simulink model "dofstuff"  (R2026b)
settings: Solver=ode4  StopTime=60  FixedStep=0.01
values from neighbouring files (symbols this model uses):
  dragCoeffVec = [CdAx;CdAy;CdAz]    [init_quadrotor.m]
  g = params.g    [QuadrotorEOM.m]    (also in QuadrotorPlant.m; init_quadrotor.m = 9.81)
  Kdtheta = 15.0    (= 15)    [init_quadrotor.m]
  Kdz = 60.0    (= 60)    [init_quadrotor.m]
  Kitheta = 5.0    (= 5)    [init_quadrotor.m]
  Kiz = 0.0    (= 0)    [init_quadrotor.m]
  Kptheta = 20.0    (= 20)    [init_quadrotor.m]
  Kpz = 150.0    (= 150)    [init_quadrotor.m]
  m = 256    [PlotAircraftSim.m]    (also in QuadrotorEOM.m = params.m; QuadrotorPlant.m = params.m; init_quadrotor.m = 5.6)
  rho = 1.225    [init_quadrotor.m]
libraries: aerolibfltsims x2, aerolibanimutils x1
settings Model: SimulationMode=accelerator  Creator=YoYo  LastModifiedBy=YoYo
settings SolverCC: MinimalZcImpactIntegration=on
settings DataIOCC: DSMLogging=off  ReturnWorkspaceOutputs=off  SaveOutput=off  SaveTime=off  SignalLogging=off
settings DebuggingCC: MultiTaskDSMMsg=none  ReadBeforeWriteMsg=DisableAll  WriteAfterReadMsg=DisableAll  WriteAfterWriteMsg=DisableAll
settings SFSimCC: SFSimEcho=off

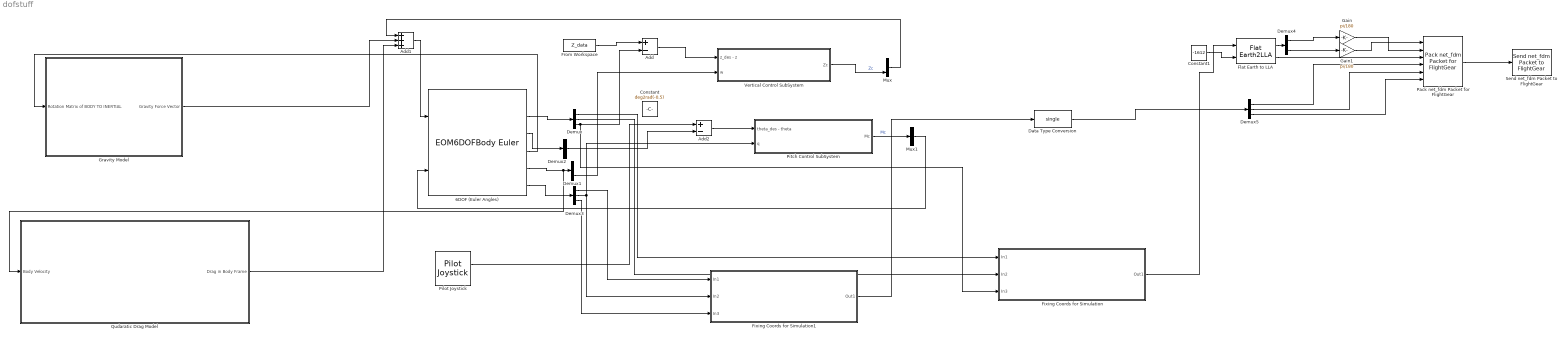
== system dofstuff ==
  6DOF (Euler Angles) : EOM6DOFBodyEuler  mass_0=5.6
  Add : Sum  Inputs=+-
  Add1 : Sum  Inputs=+++
  Add2 : Sum  Inputs=+-
  Constant : Constant  Value=deg2rad(-0.5)
  Constant1 : Constant  Value=-1612
  Data Type Conversion : DataTypeConversion  OutDataTypeStr=single  SaturateOnIntegerOverflow=off  RndMeth=Floor
  Demux{,1..3,5} (5 alike) : Demux  Outputs=3
  Demux4 : Demux  Outputs=2
  Fixing Coords for Simulation : Subsystem  Priority=-1
  Fixing Coords for Simulation1 : Subsystem  Priority=-1
  Flat Earth to LLA : FlatEarth2LLA  LL0=[40.039365 -105.226090]
  From Workspace : FromWorkspace  VariableName=Z_data
  Gain : Gain  Gain=pi/180
  Gain1 : Gain  Gain=pi/180
  Gravity Model : Subsystem
  Mux : Mux  Inputs=3
  Mux1 : Mux  Inputs=3
  Pack net_fdm Packet for FlightGear : aerolibfltsims/Pack net_fdm Packet for FlightGear  FlightGearVersion=v2019.1  ShowPositionAttitudeInputs=on  ShowVelocityAccelerationInputs=off  ShowControlSurfacePositionInputs=off  ShowEngineFuelInputs=off  ShowLandingGearInputs=off  ShowEnvironmentInputs=off  SampleTime=0.01  packetVersion=24
  Pilot Joystick : aerolibanimutils/Pilot Joystick  JoystickID=Joystick1  OutputConfiguration=FourAxis  SampleTime=0.02  action=Error
  Pitch Control SubSystem : Subsystem
  Qudaratic Drag Model : Subsystem
  Send net_fdm Packet to FlightGear : aerolibfltsims/Send net_fdm Packet to FlightGear  DestinationIpAddress=127.0.0.1  DestinationPort=5503  LocalIpPort=-1  varLen=off  SampleTime=0.01
  Vertical Control SubSystem : Subsystem
  wires:
  6DOF (Euler Angles)/2 -> Demux/1
  From Workspace/1 -> Add/1
  Demux/3 -> Fixing Coords for Simulation/3(In3), Add/2
  Add/1 -> Vertical Control SubSystem/1(z_des - z)
  6DOF (Euler Angles)/5 -> Qudaratic Drag Model/1(Body Velocity), Demux1/1
  Demux1/3 -> Vertical Control SubSystem/2(w)
  Vertical Control SubSystem/1(Zc) -> Mux/3  "Zc"
  Mux/1 -> Add1/1
  Add1/1 -> 6DOF (Euler Angles)/1
  6DOF (Euler Angles)/4 -> Gravity Model/1(Rotation Matrix of BODY TO INERTIAL)
  Gravity Model/1(Gravity Force Vector) -> Add1/2
  Qudaratic Drag Model/1(Drag in Body Frame) -> Add1/3
  6DOF (Euler Angles)/3 -> Demux2/1
  Demux2/2 -> Add2/2
  Add2/1 -> Pitch Control SubSystem/1(theta_des - theta)
  6DOF (Euler Angles)/6 -> Demux3/1
  Demux3/2 -> Fixing Coords for Simulation1/2(In2), Pitch Control SubSystem/2(q)
  Pitch Control SubSystem/1(Mc) -> Mux1/2  "Mc"
  Mux1/1 -> 6DOF (Euler Angles)/2
  Demux/1 -> Fixing Coords for Simulation/1(In1)
  Demux/2 -> Fixing Coords for Simulation/2(In2)
  Demux3/1 -> Fixing Coords for Simulation1/1(In1)
  Demux3/3 -> Fixing Coords for Simulation1/3(In3)
  Fixing Coords for Simulation/1(Out1) -> Flat Earth to LLA/1
  Pilot Joystick/2 -> Add2/1
  Constant1/1 -> Flat Earth to LLA/2
  Flat Earth to LLA/2 -> Pack net_fdm Packet for FlightGear/3
  Flat Earth to LLA/1 -> Demux4/1
  Demux5/1 -> Pack net_fdm Packet for FlightGear/4
  Demux5/2 -> Pack net_fdm Packet for FlightGear/5
  Demux5/3 -> Pack net_fdm Packet for FlightGear/6
  Pack net_fdm Packet for FlightGear/1 -> Send net_fdm Packet to FlightGear/1
  Fixing Coords for Simulation1/1(Out1) -> Data Type Conversion/1
  Data Type Conversion/1 -> Demux5/1
  Demux4/1 -> Gain/1
  Demux4/2 -> Gain1/1
  Gain/1 -> Pack net_fdm Packet for FlightGear/2
  Gain1/1 -> Pack net_fdm Packet for FlightGear/1

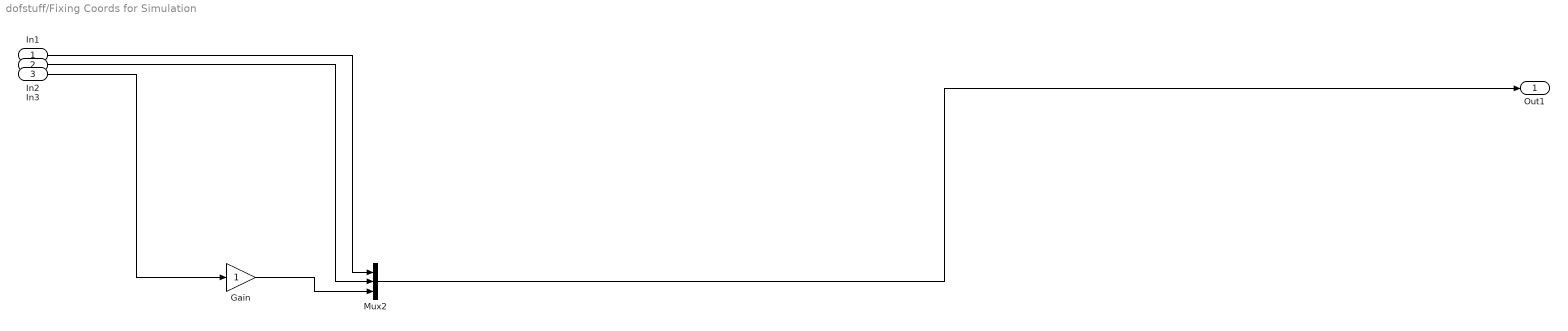
== system dofstuff/Fixing Coords for Simulation ==
  In1 : Inport
  In2 : Inport  Port=2
  In3 : Inport  Port=3
  Gain : Gain
  Mux2 : Mux  Inputs=3
  Out1 : Outport
  wires:
  Mux2/1 -> Out1/1
  In2/1 -> Mux2/2
  Gain/1 -> Mux2/3
  In1/1 -> Mux2/1
  In3/1 -> Gain/1

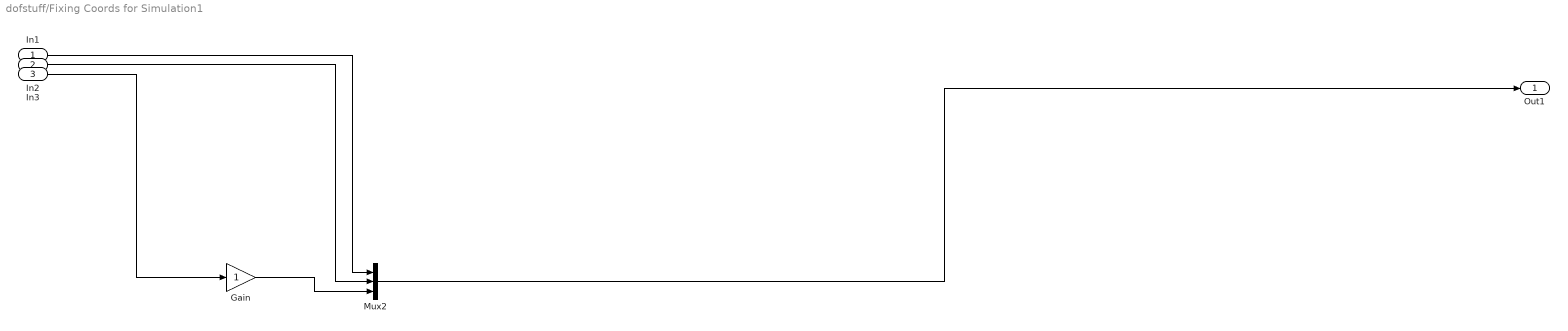
== system dofstuff/Fixing Coords for Simulation1 ==
  In1 : Inport
  In2 : Inport  Port=2
  In3 : Inport  Port=3
  Gain : Gain
  Mux2 : Mux  Inputs=3
  Out1 : Outport
  wires:
  Mux2/1 -> Out1/1
  In2/1 -> Mux2/2
  Gain/1 -> Mux2/3
  In1/1 -> Mux2/1
  In3/1 -> Gain/1

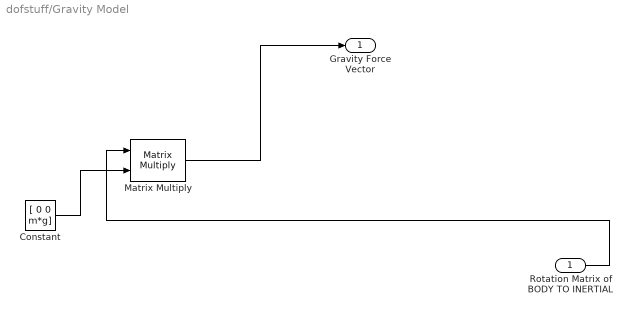
== system dofstuff/Gravity Model ==
  Rotation Matrix of BODY TO INERTIAL : Inport
  Constant : Constant  Value=[ 0 0 m*g]
  Matrix Multiply : Product  Multiplication=Matrix(*)
  Gravity Force Vector : Outport
  wires:
  Constant/1 -> Matrix Multiply/2
  Rotation Matrix of BODY TO INERTIAL/1 -> Matrix Multiply/1
  Matrix Multiply/1 -> Gravity Force Vector/1

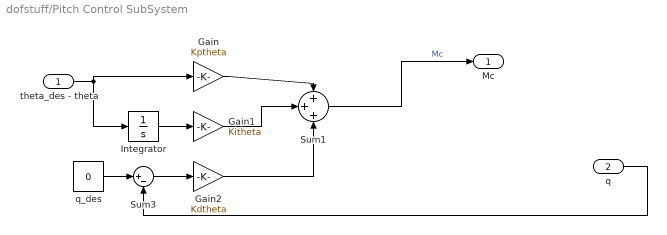
== system dofstuff/Pitch Control SubSystem ==
  theta_des - theta : Inport
  q : Inport  Port=2
  Gain : Gain  Gain=Kptheta
  Gain1 : Gain  Gain=Kitheta
  Gain2 : Gain  Gain=Kdtheta
  Integrator : Integrator  LimitOutput=on  UpperSaturationLimit=500  LowerSaturationLimit=-500
  Sum1 : Sum  Inputs=+++
  Sum3 : Sum  Inputs=|+-
  q_des : Constant  Value=0
  Mc : Outport
  wires:
  Sum1/1 -> Mc/1  "Mc"
  theta_des - theta/1 -> Integrator/1, Gain/1
  q/1 -> Sum3/2
  Gain/1 -> Sum1/1
  Sum3/1 -> Gain2/1
  Integrator/1 -> Gain1/1
  q_des/1 -> Sum3/1
  Gain1/1 -> Sum1/2
  Gain2/1 -> Sum1/3

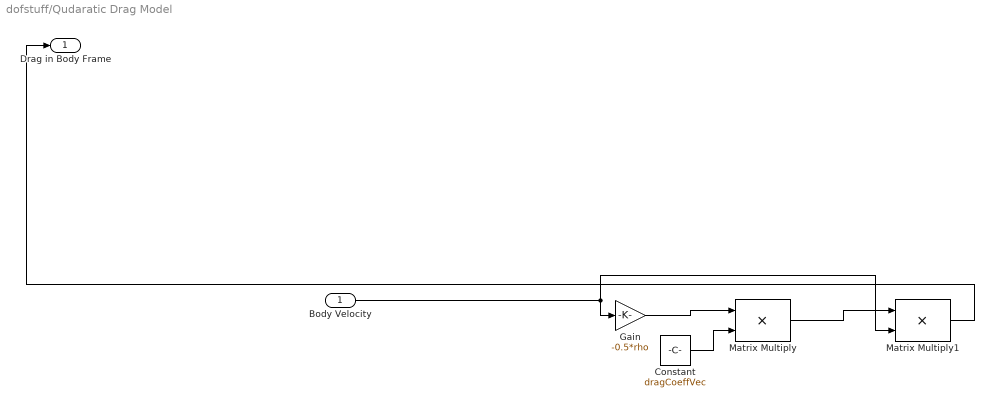
== system dofstuff/Qudaratic Drag Model ==
  Body Velocity : Inport
  Constant : Constant  Value=dragCoeffVec
  Gain : Gain  Gain=-0.5*rho
  Matrix Multiply : Product
  Matrix Multiply1 : Product
  Drag in Body Frame : Outport
  wires:
  Matrix Multiply/1 -> Matrix Multiply1/1
  Gain/1 -> Matrix Multiply/1
  Body Velocity/1 -> Gain/1, Matrix Multiply1/2
  Constant/1 -> Matrix Multiply/2
  Matrix Multiply1/1 -> Drag in Body Frame/1

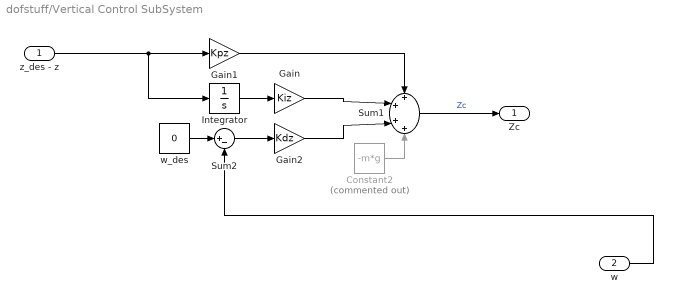
== system dofstuff/Vertical Control SubSystem ==
  z_des - z : Inport
  w : Inport  Port=2
  Constant2 : Constant  Commented=on  Value=-m*g
  Gain : Gain  Gain=Kiz
  Gain1 : Gain  Gain=Kpz
  Gain2 : Gain  Gain=Kdz
  Integrator : Integrator  LimitOutput=on  UpperSaturationLimit=500  LowerSaturationLimit=-500
  Sum1 : Sum  Inputs=++++
  Sum2 : Sum  Inputs=|+-
  w_des : Constant  Value=0
  Zc : Outport
  wires:
  w/1 -> Sum2/2
  Constant2/1 -> Sum1/4
  Gain1/1 -> Sum1/1
  Sum1/1 -> Zc/1  "Zc"
  w_des/1 -> Sum2/1
  Integrator/1 -> Gain/1
  z_des - z/1 -> Integrator/1, Gain1/1
  Sum2/1 -> Gain2/1
  Gain2/1 -> Sum1/3
  Gain/1 -> Sum1/2
